simulink model "FIR_Lowpass_Model"  (R2025a)
settings: Solver=VariableStepAuto  StartTime=0.0  StopTime=0.02  RelTol=1e-3
values from neighbouring files (symbols this model uses):
  b = [-0.000630469148644 -0.00181856812428 -0.00256194161246 -0.0015874939944 0.00236951266897 0.00833249697835 0.011803612855 0.00675929677933 -0.00917451199773 -0.029730906886 -0.0398164522664 -0.0223016476387 ... (32 elements, 1x32)]    [FIR_Lowpass_Reference.mat]    (also in FIR_Verilog_Data.mat)
undefined symbols (not defined in the file or in its folder): dspblkCoreblockFVToolHelper, gcbh
settings Model: Creator=ACER  LastModifiedBy=ACER

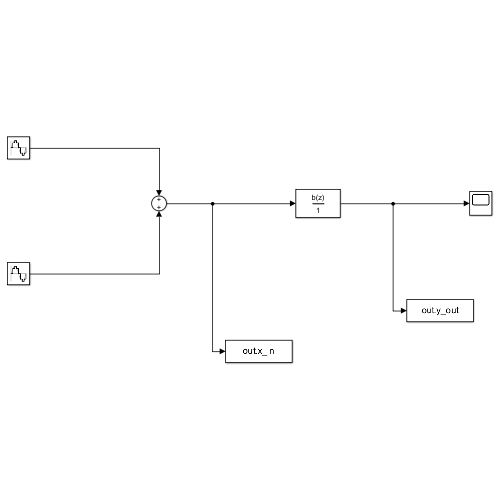
[thumbnail: Simulink's stored preview of the top-level diagram]
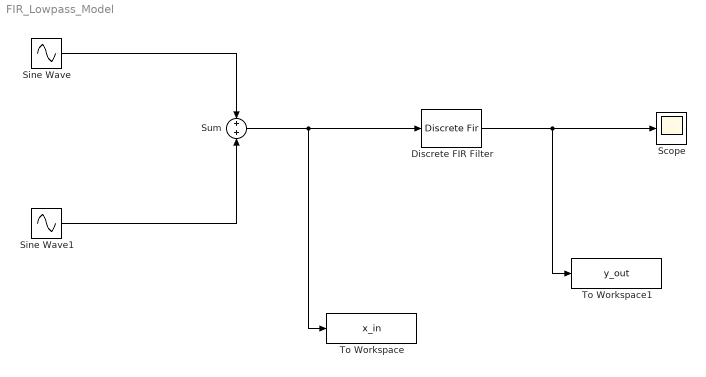
== system FIR_Lowpass_Model ==
  Discrete FIR Filter : DiscreteFir  LoadFcn=dspblkCoreblockFVToolHelper(gcbh,'load');  Coefficients=b
      settings: CopyFcn=dspblkCoreblockFVToolHelper(gcbh,'copy');  DeleteFcn=dspblkCoreblockFVToolHelper(gcbh,'close');  ModelCloseFcn=dspblkCoreblockFVToolHelper(gcbh,'close');  PreSaveFcn=dspblkCoreblockFVToolHelper(gcbh,'presave');  PostSaveFcn=dspblkCoreblockFVToolHelper(gcbh,'postsave');  CloseFcn=dspblkCoreblockFVToolHelper(gcbh,'close');
  Scope : Scope
      settings: ActiveDisplayYMinimum=-0.86468476726035837  ActiveDisplayYMaximum=0.86157918050234883
  Sine Wave : Sin  Amplitude=0.7  Frequency=2*pi*500  SampleTime=1/8000
  Sine Wave1 : Sin  Amplitude=0.5  Frequency=2*pi*2500  SampleTime=1/8000
  Sum : Sum
  To Workspace : ToWorkspace  VariableName=x_in  SaveFormat=Timeseries  SampleTime=-1
  To Workspace1 : ToWorkspace  VariableName=y_out  SaveFormat=Timeseries  SampleTime=-1
  wires:
  Sine Wave/1 -> Sum/1
  Sine Wave1/1 -> Sum/2
  Sum/1 -> To Workspace/1, Discrete FIR Filter/1
  Discrete FIR Filter/1 -> To Workspace1/1, Scope/1
